simulink model "Coding_Libraries"  (R2026b)
settings: Solver=VariableStepAuto
undefined symbols (not defined in the file): Snake_RBT
settings Model: Creator=Janelyn Anderson  LastModifiedBy=Janelyn Anderson

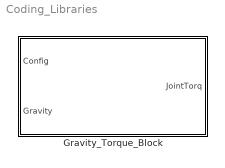
== system Coding_Libraries ==
  Gravity_Torque_Block : Subsystem  mask{RigidBodyTree=Snake_RBT, SimulateUsing=Code generation}
      mask prompts: RigidBodyTree "robotics:robotslmanip:blockmask:RigidBodyTreePrompt"; SimulateUsing "SystemBlock:MATLABSystem:SimulateUsing"
      mask init:
      | try
      |     [TreeStruct, NumBodies, sysName] = robotics.slmanip.internal.block.RBTAlgorithmBlockMasks.updateMaskWorkSpaceVariables(gcb, RigidBodyTree);
      |     robotics.slmanip.internal.block.RBTAlgorithmBlockMasks.updateBlockInputDimensions(gcb, TreeStruct,'Config');
      | catch ME
      |     TreeStruct = [];  NumBodies = [];  sysName = '???';
      |     throw(ME);
      | end
      mask TypeOptions SimulateUsing: MATLAB System1/SimulateUsing
      mask DialogControl RigidBodyTree Prompt: Rigid body tree:
      mask DialogControl SimulateUsing Prompt: Simulate using:
      mask DialogControl SimulateUsing Tooltip: SystemBlock:MATLABSystem:SimulateUsingDescription
      mask Display:
      | if (strcmp(sysName,'???'))
      |     color('red');
      | else
      |     color('blue');
      | end
      | text(0.99, 0.99, sysName, 'horizontalAlignment', 'right', 'verticalAlignment','top');
      | 
      | color('black');
      | if ~isempty(TreeStruct)
      |     g = TreeStruct.Gravity;
      | else
      |     g = [0 0 0];
      | end
      | DescText = sprintf('Gravity: [%g %g %g]',g(1),g(2),g(3));
      | text(0.5, 0.05, DescText, 'horizontalAlignment', 'center', 'verticalAlignment','bottom');
      | 
      | port_label('input', 1, 'Config')
      | port_label('input', 2, 'Gravity')
      | port_label('output', 1, 'JointTorq')

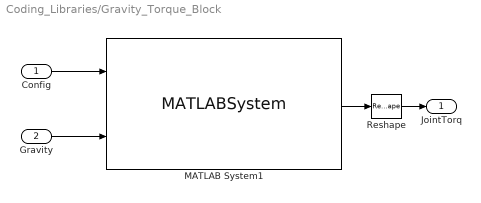
== system Coding_Libraries/Gravity_Torque_Block ==
  Config : Inport  PortDimensions=6
  Gravity : Inport  Port=2  PortDimensions=3
  MATLAB System1 : MATLABSystem  System=CustomGravityTorqueBlock  TreeStruct=TreeStruct  SimulateUsing=Code generation
      mask Type: CustomGravityTorqueBlock
  Reshape : Reshape
  JointTorq : Outport  VectorParamsAs1DForOutWhenUnconnected=off
  wires:
  Config/1 -> MATLAB System1/1
  Reshape/1 -> JointTorq/1
  MATLAB System1/1 -> Reshape/1
  Gravity/1 -> MATLAB System1/2
